simulink model "codeur_hamming"  (R2023b)
settings: Solver=FixedStepDiscrete  StartTime=0.0  StopTime=10.0  FixedStep=Tc_reg  RelTol=1e-3
values from neighbouring files (symbols this model uses):
  Tc_reg = 1    [partie4_codeur_simulink.m]    (also in partie4_decodeur_simulink.m)
libraries: simulink x3
settings Model: Creator=e2405714  LastModifiedBy=e2405714

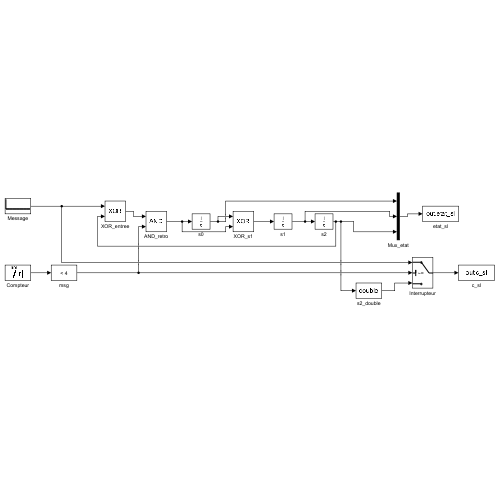
[thumbnail: Simulink's stored preview of the top-level diagram]
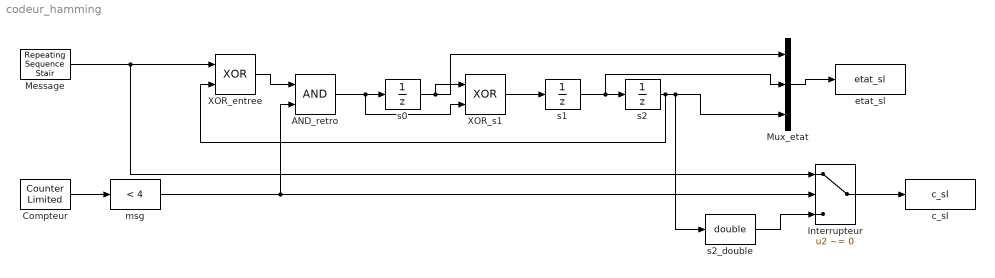
== system codeur_hamming ==
  AND_retro : Logic  AllPortsSameDT=off  OutDataTypeStr=boolean
  Compteur : simulink/Sources/Counter Limited  uplimit=6  tsamp=Tc_reg
  Interrupteur : Switch  Criteria=u2 ~= 0  SaturateOnIntegerOverflow=off  InputSameDT=off
  Message : simulink/Sources/Repeating Sequence Stair  OutValues=seq_in  tsamp=Tc_reg  OutMin=[]  OutMax=[]  OutDataTypeStr=double  OutputDataTypeScalingMode=double  OutDataType=fixdt(0,8)  ConRadixGroup=Best Precision: Vector-wise  OutScaling=2^-12
  Mux_etat : Mux  Inputs=3
  XOR_entree : Logic  Operator=XOR  AllPortsSameDT=off  OutDataTypeStr=boolean
  XOR_s1 : Logic  Operator=XOR  AllPortsSameDT=off  OutDataTypeStr=boolean
  c_sl : ToWorkspace  VariableName=c_sl  SampleTime=-1
  etat_sl : ToWorkspace  VariableName=etat_sl  SampleTime=-1
  msg : simulink/Logic and Bit Operations/Compare To Constant  relop=<  const=4  OutDataTypeStr=boolean
  s0 : UnitDelay  SampleTime=Tc_reg  HasFrameUpgradeWarning=on
  s1 : UnitDelay  SampleTime=Tc_reg  HasFrameUpgradeWarning=on
  s2 : UnitDelay  SampleTime=Tc_reg  HasFrameUpgradeWarning=on
  s2_double : DataTypeConversion  OutDataTypeStr=double  SaturateOnIntegerOverflow=off  RndMeth=Floor
  wires:
  Message/1 -> Interrupteur/1, XOR_entree/1
  Compteur/1 -> msg/1
  msg/1 -> AND_retro/2, Interrupteur/2
  XOR_entree/1 -> AND_retro/1
  AND_retro/1 -> s0/1, XOR_s1/2
  s0/1 -> XOR_s1/1, Mux_etat/1
  XOR_s1/1 -> s1/1
  s1/1 -> s2/1, Mux_etat/2
  s2/1 -> s2_double/1, Mux_etat/3, XOR_entree/2
  s2_double/1 -> Interrupteur/3
  Interrupteur/1 -> c_sl/1
  Mux_etat/1 -> etat_sl/1
